simulink model "turtlebot_test0"  (R2026a)
settings: Solver=FixedStepDiscrete  StopTime=inf  FixedStep=0.1
StartFcn:
  | 
  |  % Do not delete, this is an auto-generated function to log ROS message.
  |  ros.slros.internal.ROSUtil.loggerStartFcn(bdroot)
StopFcn:
  | 
  |  % Do not delete, this is an auto-generated function to log ROS message.
  |  ros.slros.internal.ROSUtil.logROSMessageToBagFile(bdroot);
model workspace (MAT data in the model file):
  ROSLoggingInfo_.GenBagFile = 1
  ROSLoggingInfo_.BagFileName = 'turtlebot_test0'
  ROSLoggingInfo_.CompressionFormat = 'uncompressed'
  ROSLoggingInfo_.ChunkSize = 786432
  ROSLoggingInfo_.LogOption = 'Default'
  ROSLoggingInfo_.FilePrefix = ''
  ROSLoggingReload_{1,1} = 'turtlebot_test0/Subscribe'
  ROSLoggingReload_{2,1} = 'turtlebot_test0/Blank Message'
  ROSLoggingReload_{3,1} = 'turtlebot_test0/Bus
    | Assignment'
  ROSLoggingReload_{1,2} = 0
  ROSLoggingReload_{2,2} = 0
  ROSLoggingReload_{3,2} = 0
  ROSLoggingReload_{1,3} = 'odom_subscribe'
  ROSLoggingReload_{2,3} = 'blank_message'
  ROSLoggingReload_{3,3} = 'cmd_vel_bus_assignment'
  ROSLoggingTable_ = {}
libraries: robotlib x3
settings Model: SimulationMode=external  Creator=linuxpc  LastModifiedBy=linuxpc
settings HardwareCC: ProdHWDeviceType=Generic->Unspecified (assume 32-bit Generic)  UseEmbeddedCoderFeatures=off
settings RTWCC: SystemTargetFile=ert.tlc  HardwareBoard=Robot Operating System (ROS)  TLCOptions="-aInlineSetEventsForThisBaseRateFcn=TLC_FALSE -aSuppressMultiTaskScheduler=TLC_FALSE  -aRateBasedStepFcn=0"  Toolchain=Catkin  TargetLang=C++  Description=Embedded Coder
settings ERTTargetCC: SupportNonInlinedSFcns=on

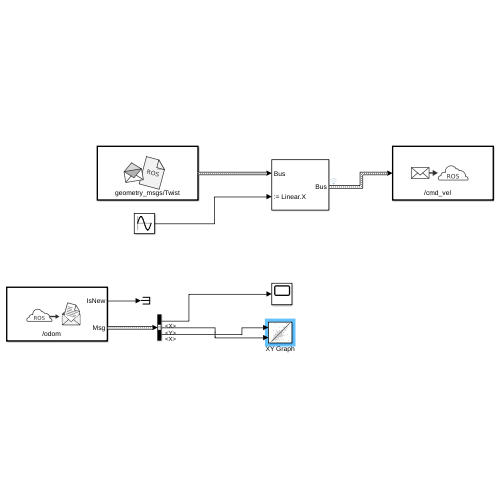
[thumbnail: Simulink's stored preview of the top-level diagram]
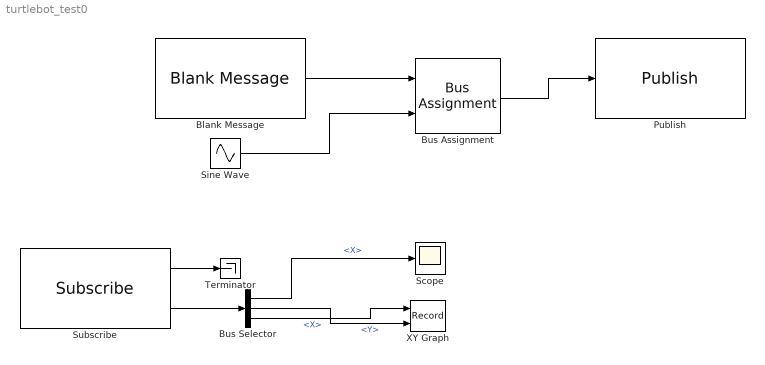
== system turtlebot_test0 ==
  Blank Message : robotlib/Blank Message  messageClass=Message  entityType=geometry_msgs/Twist  messageType=geometry_msgs/Twist  SampleTime=inf  legacyBusStruct=off
  Bus Assignment : BusAssignment  AssignedSignals=Linear.X
  Bus Selector : BusSelector  OutputSignals=Twist.Twist.Linear.X,Pose.Pose.Position.Y,Pose.Pose.Position.X
  Publish : robotlib/Publish  topicSource=Select from ROS network  topic=/cmd_vel  messageType=geometry_msgs/Twist  legacyBusStruct=off  messageQueueLength=1
  Scope : Scope
      settings: ActiveDisplayYMinimum=-0.033115839476285866  ActiveDisplayYMaximum=0.11472392347833214
  Sine Wave : Sin  Amplitude=0.05  Frequency=0.005  SampleTime=0
  Subscribe : robotlib/Subscribe  topicSource=Select from ROS network  topic=/odom  messageType=nav_msgs/Odometry  SampleTime=-1  legacyBusStruct=off  messageQueueLength=1
  Terminator : Terminator
  XY Graph : Record  NumPorts=2.0  FileSettingsInternal="{\"entries\":[{\"content\":{\"excelSettings\":{\"content\":{},\"type\":\"Streamout.ExcelSettings\"},\"parquetSettings\":{\"content\":{},\"type\":\"Streamout.ParquetSettings\"}},\"type\":\"Streamout.FileSettingStorage\",\"uuid\":\"\"}],\"packageUris\":[\"http:\\/\\/schema.mathworks.com\\/mf0\\/streamout_blocks\\/R2020a\"],\"version\":\"1.0\"}"  FrameSettings=[0, 0]  Layout=[1 1]  SignalsInternal="{\"entries\":[{\"content\":{\"signals\":[{\"content\":{\"blockPath\":[],\"dimensions\":[1],\"domain\":\"\",\"lineColor\":\"#a2142f\",\"plots\":[ 1 ],\"port\":1,\"sid\":[\"\"],\"signalID\":1,\"signalName\":\"<X>\"},\"type\":\"RecordBlkView.Signal\",\"uuid\":\"\"},{\"content\":{\"blockPath\":[],\"dimensions\":[1],\"domain\":\"\",\"lineColor\":\"#139fff\",\"plots\":[ 1 ],\"port\":2,\"sid\":[\"\"],\"signalID\":2,\"signalName\":\"<Y>\"},\"type\":\"RecordBlkView.Signal\",\"uuid\":\"\"}]},\"type\":\"RecordBlkView.InputSignals\",\"uuid\":\"\"}],\"packageUris\":[\"http:\\/\\/schema.mathworks.com\\/mf0\\/streamout_blocks\\/R2020a\"],\"version\":\"1.0\"}"  VisualizationBindings="{\"xyplotplugin\":{\"info\":[{\"series\":[{\"bindingParametersList\":[{\"parameter\":\"X-Axis\",\"signalID\":1,\"signalName\":\"<X>\"},{\"parameter\":\"Y-Axis\",\"signalID\":2,\"signalName\":\"<Y>\"}],\"seriesID\":0}],\"subplotID\":1}]}}"  CompatibilityTag=XY
  wires:
  Blank Message/1 -> Bus Assignment/1
  Bus Assignment/1 -> Publish/1
  Sine Wave/1 -> Bus Assignment/2
  Bus Selector/1 -> Scope/1  "<X>"
  Subscribe/1 -> Terminator/1
  Subscribe/2 -> Bus Selector/1
  Bus Selector/2 -> XY Graph/2  "<Y>"
  Bus Selector/3 -> XY Graph/1  "<X>"
